simulink model "lab1_square_2d"  (R2025b)
settings: Solver=ode4  StartTime=0.0  StopTime=13  FixedStep=0.01  RelTol=1e-3
model workspace (MAT data in the model file):
  SIDE = 2
  SPEED = 1
  TRACK = 0.3
  TURN_RATE = 1.57079632679
  WHEEL_ERROR = 0
  WHEEL_RADIUS = 0.05
libraries: robotmobilelib x1
settings Model: Creator=xion  LastModifiedBy=xion

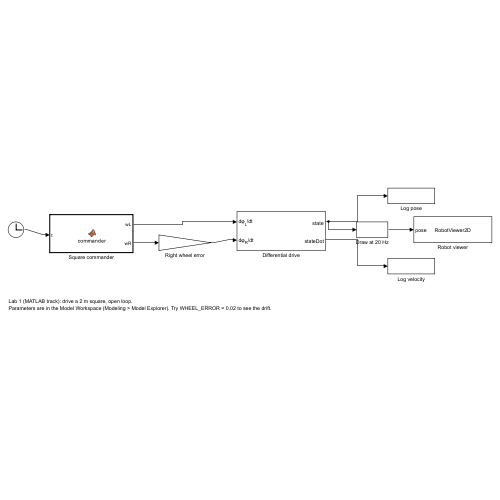
[thumbnail: Simulink's stored preview of the top-level diagram]
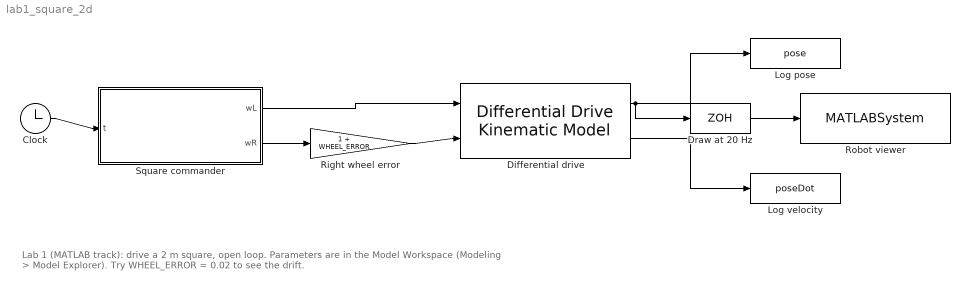
== system lab1_square_2d ==
  note: Lab 1 (MATLAB track): drive a 2 m square, open loop.
      | Parameters are in the Model Workspace (Modeling > Model Explorer). Try WHEEL_ERROR = 0.02 to see the drift.
  Clock : Clock
  Differential drive : robotmobilelib/Differential Drive Kinematic Model  VehicleInputs=Wheel Speeds  WheelRadius=WHEEL_RADIUS  WheelSpeedRange=[-inf inf]  TrackWidth=TRACK  InitialState=[0; 0; 0]  SimulateUsing=Interpreted execution
  Draw at 20 Hz : ZeroOrderHold  SampleTime=0.05
  Log pose : ToWorkspace  VariableName=pose  SampleTime=-1
  Log velocity : ToWorkspace  VariableName=poseDot  SampleTime=-1
  Right wheel error : Gain  Gain=1 + WHEEL_ERROR
  Robot viewer : MATLABSystem  System=RobotViewer2D  Side=SIDE  SimulateUsing=Interpreted execution
      mask Type: RobotViewer2D
  Square commander : MATLAB Function  TreatAsAtomicUnit=on
  wires:
  Clock/1 -> Square commander/1(t)
  Square commander/1(wL) -> Differential drive/1
  Square commander/2(wR) -> Right wheel error/1
  Right wheel error/1 -> Differential drive/2
  Differential drive/1 -> Log pose/1, Draw at 20 Hz/1
  Differential drive/2 -> Log velocity/1
  Draw at 20 Hz/1 -> Robot viewer/1

== matlab function lab1_square_2d/Square commander ==
  data: t input; wL output; wR output; SIDE parameter; SPEED parameter; TURN_RATE parameter; WHEEL_RADIUS parameter; TRACK parameter
function [wL, wR] = commander(t, SIDE, SPEED, TURN_RATE, WHEEL_RADIUS, TRACK)
% Open-loop square, as in the Python lab: drive SIDE metres, turn 90 degrees left,
% four times, then stop. No sensor is used: the robot does not know where it is.
tSide = SIDE / SPEED;            % time to drive one side, s
tTurn = (pi/2) / TURN_RATE;      % time to turn 90 degrees, s
period = tSide + tTurn;
if t >= 4 * period
    v = 0; w = 0;                % finished: stop
elseif mod(t, period) < tSide
    v = SPEED; w = 0;            % drive forward
else
    v = 0; w = TURN_RATE;        % turn left on the spot
end
% Inverse kinematics of a differential drive: body speeds -> wheel speeds (rad/s)
wL = (v - w * TRACK / 2) / WHEEL_RADIUS;
wR = (v + w * TRACK / 2) / WHEEL_RADIUS;
